simulink library "myLib"  (R2024b)
settings: Solver=VariableStepAuto  StartTime=0.0  StopTime=10.0  RelTol=1e-3
undefined symbols (not defined in the file or in its folder): SampleTime
libraries: $bdroot x6, mcbcontrolslib x1
settings Model: Creator=sakee  LastModifiedBy=sakee

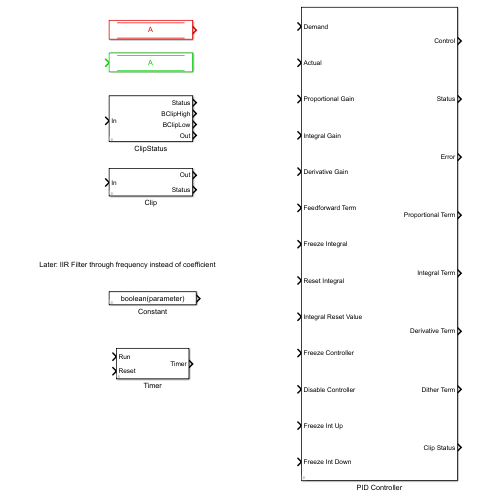
[thumbnail: Simulink's stored preview of the top-level diagram]
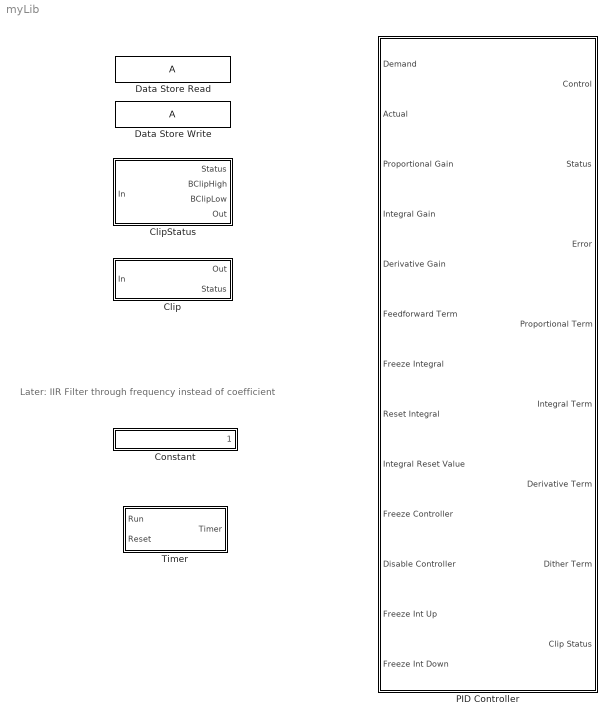
== system myLib ==
  note: Later: IIR Filter through frequency instead of coefficient
  Clip : Subsystem  mask{Upper=0, Lower=0}
  ClipStatus : Subsystem  mask{Upper=0, Lower=0}
  Constant : Subsystem  mask{constValue=parameter, DataType=boolean}
      mask prompts: constValue "Constant"; DataType "Data Type"
      mask TypeOptions DataType: boolean | single | double | uint32 | int32 | uint16 | int16 | uint8 | int8
      mask Display: disp([DataType, '(', num2str(constValue), ')'])
  Data Store Read : DataStoreRead  IndexOptions=Index vector (dialog)  Indices=1  OutputSizes=1
  Data Store Write : DataStoreWrite  IndexOptions=Index vector (dialog)  Indices=1  OutputSizes=1
  PID Controller : Subsystem  mask{ProportionalClipHigh=0, ProportionalClipLow=0, FilterCoefficient=0.001, SampleTime=SampleTime, DerivativeClipHigh=0, DerivativeClipLow=0, LivebandMax=0, LivebandMin=0, DeadbandMax=0, DeadbandMin=0, IntegralClipHigh=0, IntegralClipLow=0}
      mask prompts: ProportionalClipHigh "Proportional Clip High"; ProportionalClipLow "Proportional Clip Low"; FilterCoefficient "IIR Filter Coefficient"; SampleTime "Sample Time"; DerivativeClipHigh "Derivative Clip High"; DerivativeClipLow "Derivative Clip Low"; LivebandMax "Liveband Max"; LivebandMin "Liveband Min"; DeadbandMax "Deadband Max"; DeadbandMin "Deadband Min"; IntegralClipHigh "Integral Clip High"; IntegralClipLow "Integral Clip Low"
  Timer : Subsystem  mask{tSampleTime=0}
      mask prompts: tSampleTime "Sample Time"
      mask DialogControl SampleTime Prompt: Sample Time

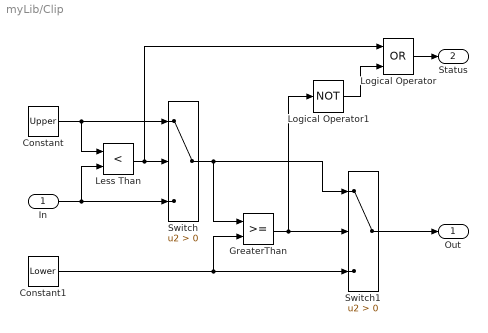
== system myLib/Clip ==
  In : Inport
  Constant : Constant  Value=Upper
  Constant1 : Constant  Value=Lower
  GreaterThan : RelationalOperator  OutDataTypeStr=boolean  RndMeth=Simplest  InputSameDT=off
  Less Than : RelationalOperator  Operator=<  OutDataTypeStr=boolean  RndMeth=Simplest  InputSameDT=off
  Logical Operator : Logic  Operator=OR  AllPortsSameDT=off  OutDataTypeStr=boolean
  Logical Operator1 : Logic  Operator=NOT  AllPortsSameDT=off  OutDataTypeStr=boolean
  Switch : Switch  Criteria=u2 > Threshold  SaturateOnIntegerOverflow=off  InputSameDT=off
  Switch1 : Switch  Criteria=u2 > Threshold  SaturateOnIntegerOverflow=off  InputSameDT=off
  Out : Outport
  Status : Outport  Port=2
  wires:
  Constant/1 -> Switch/1, Less Than/1
  In/1 -> Switch/3, Less Than/2
  Logical Operator1/1 -> Logical Operator/2
  Switch/1 -> GreaterThan/1, Switch1/1
  GreaterThan/1 -> Logical Operator1/1, Switch1/2
  Less Than/1 -> Logical Operator/1, Switch/2
  Logical Operator/1 -> Status/1
  Switch1/1 -> Out/1
  Constant1/1 -> GreaterThan/2, Switch1/3

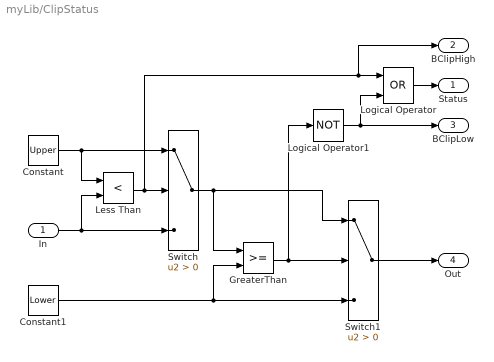
== system myLib/ClipStatus ==
  In : Inport
  Constant : Constant  Value=Upper
  Constant1 : Constant  Value=Lower
  GreaterThan : RelationalOperator  OutDataTypeStr=boolean  RndMeth=Simplest  InputSameDT=off
  Less Than : RelationalOperator  Operator=<  OutDataTypeStr=boolean  RndMeth=Simplest  InputSameDT=off
  Logical Operator : Logic  Operator=OR  AllPortsSameDT=off  OutDataTypeStr=boolean
  Logical Operator1 : Logic  Operator=NOT  AllPortsSameDT=off  OutDataTypeStr=boolean
  Switch : Switch  Criteria=u2 > Threshold  SaturateOnIntegerOverflow=off  InputSameDT=off
  Switch1 : Switch  Criteria=u2 > Threshold  SaturateOnIntegerOverflow=off  InputSameDT=off
  Status : Outport
  BClipHigh : Outport  Port=2
  BClipLow : Outport  Port=3
  Out : Outport  Port=4
  wires:
  Less Than/1 -> BClipHigh/1, Logical Operator/1, Switch/2
  In/1 -> Switch/3, Less Than/2
  Constant/1 -> Switch/1, Less Than/1
  GreaterThan/1 -> Logical Operator1/1, Switch1/2
  Constant1/1 -> GreaterThan/2, Switch1/3
  Switch/1 -> GreaterThan/1, Switch1/1
  Switch1/1 -> Out/1
  Logical Operator/1 -> Status/1
  Logical Operator1/1 -> BClipLow/1, Logical Operator/2

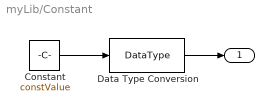
== system myLib/Constant ==
  Constant : Constant  Value=constValue
  Data Type Conversion : DataTypeConversion  OutDataTypeStr=DataType  SaturateOnIntegerOverflow=off  RndMeth=Floor
  " " : Outport
  wires:
  Constant/1 -> Data Type Conversion/1
  Data Type Conversion/1 -> " "/1

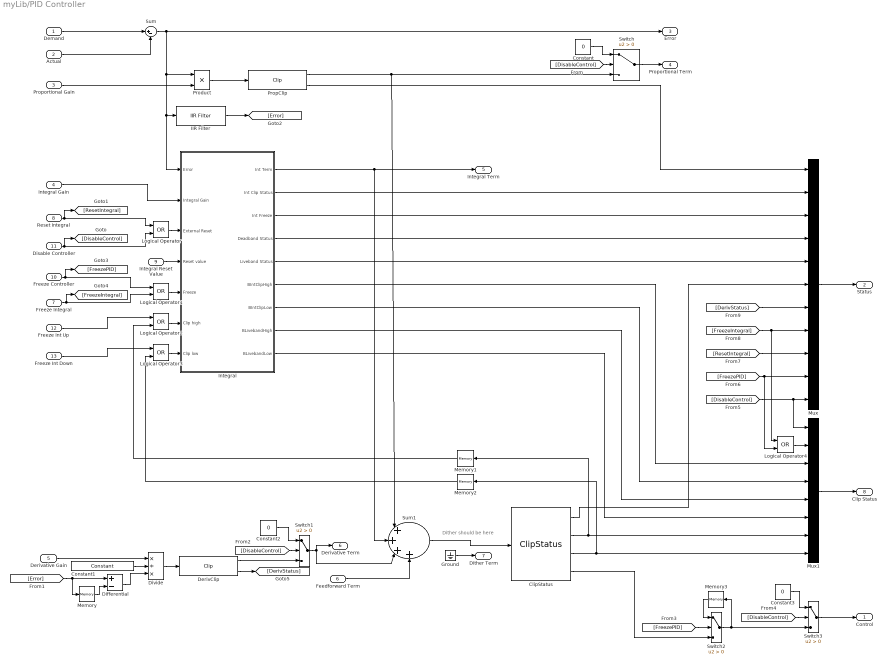
== system myLib/PID Controller ==
  note: Dither should be here
  Demand : Inport
  Actual : Inport  Port=2
  Proportional Gain : Inport  Port=3
  Integral Gain : Inport  Port=4
  Derivative Gain : Inport  Port=5
  Feedforward Term : Inport  Port=6
  Freeze Integral : Inport  Port=7
  Reset Integral : Inport  Port=8
  Integral Reset Value : Inport  Port=9
  Freeze Controller : Inport  Port=10
  "Disable Controller " : Inport  Port=11
  Freeze Int Up : Inport  Port=12
  Freeze Int Down : Inport  Port=13
  ClipStatus : $bdroot/ClipStatus  Upper=0  Lower=0
  Constant : Constant  Value=0
  Constant1 : $bdroot/Constant  constValue=SampleTime  DataType=double
  Constant2 : Constant  Value=0
  Constant3 : Constant  Value=0
  DerivClip : $bdroot/Clip  Upper=DerivativeClipHigh  Lower=DerivativeClipLow
  Differential : Sum  Inputs=+-
  Divide : Product  Inputs=*/*
  Ground : Ground
  IIR Filter : mcbcontrolslib/IIR Filter  VariantControl=Low Pass Filter  VariantSelect=Low-pass  FilterConstantInputType=Specify via dialog  Filter_constant=FilterCoefficient  advancedSettings=on  Ts=50e-6  cutOff_freq=3.1863
      settings: LibrarySourceBlock=mcbhdllib/Signal Management/IIR Filter
  Integral : Subsystem
  Logical Operator{,1..4} (5 alike) : Logic  Operator=OR  AllPortsSameDT=off  OutDataTypeStr=boolean
  Memory{,1..3} (4 alike) : Memory
  Mux : Mux  Inputs=11
  Mux1 : Mux  Inputs=8
  Product : Product
  PropClip : $bdroot/Clip  Upper=ProportionalClipHigh  Lower=ProportionalClipLow
  Sum : Sum  Inputs=|+-
  Sum1 : Sum  Inputs=|++++
  Switch{,1..3} (4 alike) : Switch  Criteria=u2 > Threshold  SaturateOnIntegerOverflow=off  InputSameDT=off
  Control : Outport
  Status : Outport  Port=2
  Error : Outport  Port=3
  Proportional Term : Outport  Port=4
  Integral Term : Outport  Port=5
  Derivative Term : Outport  Port=6
  Dither Term : Outport  Port=7
  Clip Status : Outport  Port=8
  wires:
  Demand/1 -> Sum/1
  Actual/1 -> Sum/2
  Sum/1 -> Integral/1(Error), IIR Filter/1, Product/1, Error/1
  Proportional Gain/1 -> Product/2
  "Disable Controller "/1 -> Logical Operator/2, [DisableControl]
  Switch/1 -> Proportional Term/1
  [DisableControl] -> Switch/2
  Constant/1 -> Switch/1
  Product/1 -> PropClip/1
  PropClip/1 -> Switch/3, Sum1/1
  IIR Filter/1 -> [Error]
  Constant1/1 -> Divide/2
  Derivative Gain/1 -> Divide/1
  [Error] -> Memory/1, Differential/1
  Differential/1 -> Divide/3
  Memory/1 -> Differential/2
  Divide/1 -> DerivClip/1
  Constant2/1 -> Switch1/1
  [DisableControl] -> Switch1/2
  DerivClip/1 -> Switch1/3
  Switch1/1 -> Derivative Term/1, Sum1/3
  Feedforward Term/1 -> Sum1/4
  Integral/1(Int Term) -> Integral Term/1, Sum1/2
  Integral Gain/1 -> Integral/2(Integral Gain)
  Logical Operator/1 -> Integral/3(External Reset)
  Reset Integral/1 -> Logical Operator/1, [ResetIntegral]
  Integral Reset Value/1 -> Integral/4(Reset value)
  Logical Operator1/1 -> Integral/5(Freeze)
  Freeze Controller/1 -> [FreezePID], Logical Operator1/1
  Freeze Integral/1 -> [FreezeIntegral], Logical Operator1/2
  Logical Operator2/1 -> Integral/6(Clip high)
  Logical Operator3/1 -> Integral/7(Clip low)
  Freeze Int Up/1 -> Logical Operator2/1
  Freeze Int Down/1 -> Logical Operator3/1
  Sum1/1 -> ClipStatus/1
  ClipStatus/2 -> Mux1/7, Memory1/1
  ClipStatus/3 -> Memory2/1, Mux1/8
  Memory1/1 -> Logical Operator2/2
  Memory2/1 -> Logical Operator3/2
  [FreezePID] -> Switch2/2
  Switch2/1 -> Memory3/1, Switch3/3
  Memory3/1 -> Switch2/1
  ClipStatus/4 -> Switch2/3
  [DisableControl] -> Switch3/2
  Constant3/1 -> Switch3/1
  Switch3/1 -> Control/1
  Ground/1 -> Dither Term/1
  Mux/1 -> Status/1
  PropClip/2 -> Mux/1
  Integral/2(Int Clip Status) -> Mux/2
  Integral/3(Int Freeze) -> Mux/3
  Integral/4(Deadband Status) -> Mux/4
  Integral/5(Liveband Status) -> Mux/5
  ClipStatus/1 -> Mux/6
  Mux1/1 -> Clip Status/1
  [FreezeIntegral] -> Mux/8, Logical Operator4/1
  [ResetIntegral] -> Mux/9
  [FreezePID] -> Logical Operator4/2, Mux/10
  [DisableControl] -> Mux/11, Mux1/1
  DerivClip/2 -> [DerivStatus]
  [DerivStatus] -> Mux/7
  Logical Operator4/1 -> Mux1/2
  Integral/6(BIntClipHigh) -> Mux1/3
  Integral/7(BIntClipLow) -> Mux1/4
  Integral/8(BLivebandHigh) -> Mux1/5
  Integral/9(BLivebandLow) -> Mux1/6

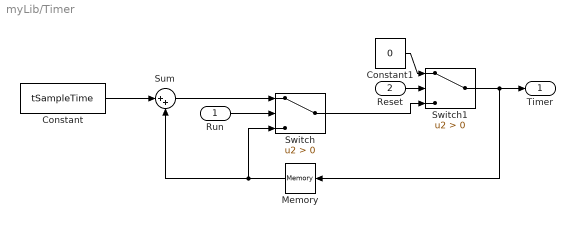
== system myLib/Timer ==
  Run : Inport
  Reset : Inport  Port=2
  Constant : Constant  Value=tSampleTime
  Constant1 : Constant  Value=0
  Memory : Memory  InheritSampleTime=on
  Sum : Sum  Inputs=|++
  Switch : Switch  Criteria=u2 > Threshold  SaturateOnIntegerOverflow=off  InputSameDT=off
  Switch1 : Switch  Criteria=u2 > Threshold  SaturateOnIntegerOverflow=off  InputSameDT=off
  Timer : Outport
  wires:
  Constant/1 -> Sum/1
  Run/1 -> Switch/2
  Sum/1 -> Switch/1
  Switch/1 -> Switch1/3
  Reset/1 -> Switch1/2
  Constant1/1 -> Switch1/1
  Switch1/1 -> Memory/1, Timer/1
  Memory/1 -> Switch/3, Sum/2

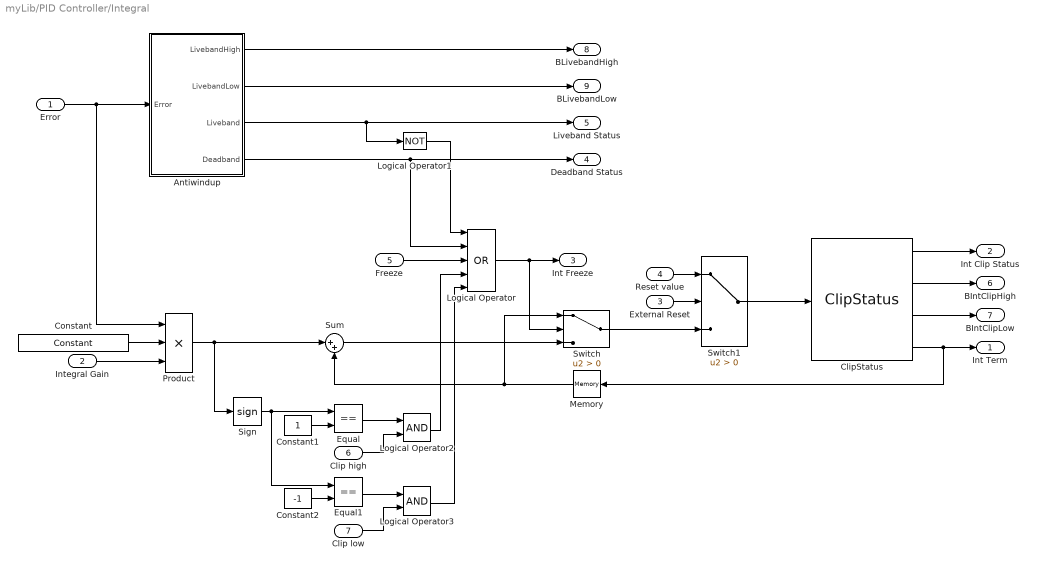
== system myLib/PID Controller/Integral ==
  Error : Inport
  Integral Gain : Inport  Port=2
  External Reset : Inport  Port=3
  Reset value : Inport  Port=4
  Freeze : Inport  Port=5
  Clip high : Inport  Port=6
  Clip low : Inport  Port=7
  Antiwindup : Subsystem  mask{LivebandMax=LivebandMax, LivebandMin=LivebandMin, DeadbandMax=DeadbandMax, DeadbandMin=DeadbandMin}
      mask prompts: LivebandMax "Liveband Max"; LivebandMin "Liveband Min"; DeadbandMax "Deadband Max"; DeadbandMin "Deadband Min"
  ClipStatus : $bdroot/ClipStatus  Upper=IntegralClipHigh  Lower=IntegralClipLow
  Constant : $bdroot/Constant  constValue=SampleTime  DataType=boolean
  Constant1 : Constant
  Constant2 : Constant  Value=-1
  Equal : RelationalOperator  Operator===  OutDataTypeStr=boolean  RndMeth=Simplest  InputSameDT=off
  Equal1 : RelationalOperator  Operator===  OutDataTypeStr=boolean  RndMeth=Simplest  InputSameDT=off
  Logical Operator : Logic  Operator=OR  Inputs=5  AllPortsSameDT=off  OutDataTypeStr=boolean
  Logical Operator1 : Logic  Operator=NOT  AllPortsSameDT=off  OutDataTypeStr=boolean
  Logical Operator2 : Logic  AllPortsSameDT=off  OutDataTypeStr=boolean
  Logical Operator3 : Logic  AllPortsSameDT=off  OutDataTypeStr=boolean
  Memory : Memory
  Product : Product  Inputs=3
  Sign : Signum
  Sum : Sum  Inputs=|++
  Switch : Switch  Criteria=u2 > Threshold  SaturateOnIntegerOverflow=off  InputSameDT=off
  Switch1 : Switch  Criteria=u2 > Threshold  SaturateOnIntegerOverflow=off  InputSameDT=off
  Int Term : Outport
  Int Clip Status : Outport  Port=2
  Int Freeze : Outport  Port=3
  Deadband Status : Outport  Port=4
  Liveband Status : Outport  Port=5
  BIntClipHigh : Outport  Port=6
  BIntClipLow : Outport  Port=7
  BLivebandHigh : Outport  Port=8
  BLivebandLow : Outport  Port=9
  wires:
  Error/1 -> Antiwindup/1(Error), Product/1
  Antiwindup/1(LivebandHigh) -> BLivebandHigh/1
  Antiwindup/2(LivebandLow) -> BLivebandLow/1
  Antiwindup/3(Liveband) -> Logical Operator1/1, Liveband Status/1
  Antiwindup/4(Deadband) -> Logical Operator/2, Deadband Status/1
  Logical Operator1/1 -> Logical Operator/1
  Freeze/1 -> Logical Operator/3
  Constant/1 -> Product/2
  Integral Gain/1 -> Product/3
  Product/1 -> Sum/1, Sign/1
  Constant1/1 -> Equal/2
  Sign/1 -> Equal1/1, Equal/1
  Constant2/1 -> Equal1/2
  Equal/1 -> Logical Operator2/1
  Equal1/1 -> Logical Operator3/1
  Clip low/1 -> Logical Operator3/2
  Clip high/1 -> Logical Operator2/2
  Logical Operator2/1 -> Logical Operator/4
  Logical Operator3/1 -> Logical Operator/5
  Sum/1 -> Switch/3
  Logical Operator/1 -> Int Freeze/1, Switch/2
  Switch/1 -> Switch1/3
  External Reset/1 -> Switch1/2
  Reset value/1 -> Switch1/1
  Switch1/1 -> ClipStatus/1
  Memory/1 -> Switch/1, Sum/2
  ClipStatus/4 -> Int Term/1, Memory/1
  ClipStatus/1 -> Int Clip Status/1
  ClipStatus/2 -> BIntClipHigh/1
  ClipStatus/3 -> BIntClipLow/1

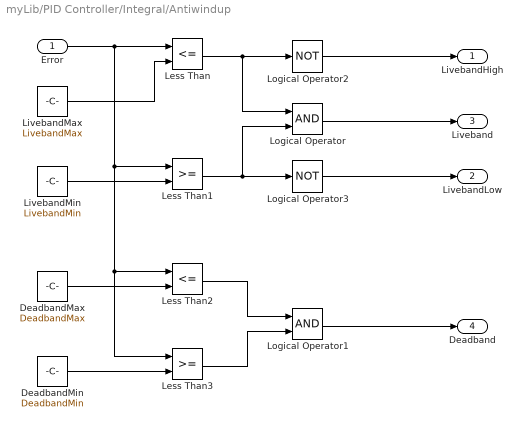
== system myLib/PID Controller/Integral/Antiwindup ==
  Error : Inport
  DeadbandMax : Constant  Value=DeadbandMax
  DeadbandMin : Constant  Value=DeadbandMin
  Less Than : RelationalOperator  Operator=<=  OutDataTypeStr=boolean  RndMeth=Simplest  InputSameDT=off
  Less Than1 : RelationalOperator  OutDataTypeStr=boolean  RndMeth=Simplest  InputSameDT=off
  Less Than2 : RelationalOperator  Operator=<=  OutDataTypeStr=boolean  RndMeth=Simplest  InputSameDT=off
  Less Than3 : RelationalOperator  OutDataTypeStr=boolean  RndMeth=Simplest  InputSameDT=off
  LivebandMax : Constant  Value=LivebandMax
  LivebandMin : Constant  Value=LivebandMin
  Logical Operator : Logic  AllPortsSameDT=off  OutDataTypeStr=boolean
  Logical Operator1 : Logic  AllPortsSameDT=off  OutDataTypeStr=boolean
  Logical Operator2 : Logic  Operator=NOT  AllPortsSameDT=off  OutDataTypeStr=boolean
  Logical Operator3 : Logic  Operator=NOT  AllPortsSameDT=off  OutDataTypeStr=boolean
  LivebandHigh : Outport
  LivebandLow : Outport  Port=2
  Liveband : Outport  Port=3
  Deadband : Outport  Port=4
  wires:
  Error/1 -> Less Than3/1, Less Than2/1, Less Than1/1, Less Than/1
  LivebandMax/1 -> Less Than/2
  LivebandMin/1 -> Less Than1/2
  DeadbandMax/1 -> Less Than2/2
  DeadbandMin/1 -> Less Than3/2
  Less Than/1 -> Logical Operator2/1, Logical Operator/1
  Less Than1/1 -> Logical Operator3/1, Logical Operator/2
  Logical Operator/1 -> Liveband/1
  Less Than2/1 -> Logical Operator1/1
  Less Than3/1 -> Logical Operator1/2
  Logical Operator1/1 -> Deadband/1
  Logical Operator3/1 -> LivebandLow/1
  Logical Operator2/1 -> LivebandHigh/1
